simulink model "BimanualCarvingModifiedSnapshot"  (R2013a)
settings: Solver=ode4  SolverMode=SingleTasking  StartTime=0.0  StopTime=inf  FixedStep=0.0005  RelTol=1e-3
StartFcn:
  |  warndlg('Dexterit-E models cannot run under simulation. Please compile your model and run it from within Dexterit-E.');set_param(bdroot,'SimulationCommand','stop')
model workspace (MAT data in the model file):
  BKIN_STEP_TIME = 0.0005
  col_x = 1
  col_y = 2
  WIDTH = 3
  HEIGHT = 4
  TARGET_COL = 1
  LOAD = 2
  TRAJ_DURATION_COL = 3
  MAX_LOAD = 2
  FORCE_ON = 1
  HAND_RADIUS = 6
  REST_COL = 4
  TRAINING_COL = 5
  HAND_COLOR = 5
  TARGET_STROKE = 8
  TARGET_RADIUS = 9
  xMaxCursor = 15
  yMaxCursor = 16
  TARGET_COLOR = 7
  START_X = 10
  START_Y = 11
  STIFFNESS_MATERIAL = 3
  MATERIAL_MASS = 4
  MATERIAL_DAMPING = 5
  STIFFNESS_HANDS = 6
  MATERIAL_GOAL_COLOR = 12
  SCALE_VIBRATION = 7
  STONE_WIDTH = 6
  MATERIAL_DUCTILITY = 8
  TARG_COLOR = 1
  TEXT_COLOR = 13
  TEXTBOX_WIDTH = 14
  TEXTBOX_HEIGHT = 15
  ROTATION = 16
  LABEL_TEXT = 17
  LABEL_COLOR = 18
  LABEL_HEIGHT = 19
  ADVANCE_EMG_PLACEMENT = 2
  ADVANCE_EMG_MAX = 3
  EMG_ADVANCE_BUTTON = 1
  EMG_MVC_BUTTON = 2
  START_TRIAL = 3
  END_TRIAL = 4
  MUSC_NUM = 2
  HAND_DISTANCE = 3
  SYN_NUM = 4
undefined symbols (not defined in the file or in its folder): slselsubs
libraries: xpclib x9, simulink x6, General x3, KINARM_loads x2, Video x2, KINARM_IO x1, KINARM_EP_loads x1
(part 3 of 6)

== matlab function BimanualCarvingModifiedSnapshot/Draw_Hand_Endpoint/MATLAB Function ==
  data: target input; VCODE output; state_in input; target_type input; opacity_in input; target_display input; x_index input; y_index input; num_states input; stateindices input; target_labels input; KINData input; trial_state input
function VCODE = fcn(target, state_in, target_type, opacity_in, target_display, x_index, y_index, num_states, stateindices, target_labels, KINData, trial_state)

% stateindices should follow this order (depending on target-type):
% 1: length of tool (m)
% 2: stroke colour
% 3: stroke width
% 4: major radius / radius / start point (line)
% 5: minor radius / end point (line)
% 6: orientation angle



% VCODEs are length 70. All units in a VCODE should be SI, e.g. (m) and (rad). Elements in a VCODE are defined as follows:
%
% For all target types:
%  1: target type
%       1 - circle
%       2 - ellipse
%       3 - rectangle
%       4 - line
%       5 - triangle
%       11 - circle with label
%       12 - ellipse with label
%       13 - rectangle with label
%       14 - line with label
%       15 - triangle with label
%  2: target on/off status and target display (which display target will appear on)
%		0 - off
%		1 - on, appearing on both subject and operator displays
%       2 - on, appearing on subject display only
%       3 - on, appearing on operator display only
%  3: x position (m)
%  4: y position (m)
%  5: fill colour (RRGGBB) or texture index
%  6: stroke colour (RRGGBB) or texture index
%  7: stroke width
%  8: reserved for target background ID
%  9: opacity
%
% For circles:
%  10: radius (m)
%
% For ellipses:
%  10: major radius (m)
%  11: minor radius (m)
%  12: orientation of major axis (rad)
%
% For rectangles:
%  10: length (m)
%  11: height (m)
%  12: orientation (rad) (relative to x, y already shown)
%
% For lines:
%  10: endpoint x-axis coordinate relative to start point (m)
%  11: endpoint y-axis coordinate relative to start point (m)
%
% For triangles:
%  10: length (m)
%  11: height (m)
%  12: offset of peak from midpoint of length (m)
%  13: orientation (rad)
%
% For all labelled target types:
%  14: reserved
%  15-64: label characters (indexes in ISO 8859-1 character set)
%  65: label colour (0xRRGGBB), opacity is set by the vcode's opacity (9).
%  66: label height (m)
%  67: reserved
%  68: reserved
%  69: reserved
%  70: reserved

num_targets = 2;

% NOTE: we assume that the STATE and/or OPACITY inputs are vectors. 

% If the length of the input STATE is not the same as the number of targets then make STATE a column vector of the same length as 
% the TARGET input, using the first STATE (i.e. all targets get the same state) 
if num_targets == length(state_in)
	state = reshape(state_in, num_targets, 1);
else
	state = state_in(1) * ones(num_targets, 1);
end


% If the length of the input OPACITY is not the same as the number of targets then make OPACITY a column vector of the same length as
% the TARGET input, using the first OPACITY (i.e. all targets get the same opacity) 
if num_targets == length(opacity_in)
	opacity = reshape(opacity_in, num_targets, 1);
else
	opacity = opacity_in(1) * ones(num_targets, 1);
end


% Clamping the opacity to [0, 100].
opacity = min(opacity, 100);
opacity = max(opacity, 0);

VCODE = zeros(num_targets, 70);

% Set the target type. Targets with labels have type codes 10 greater than their unlabelled counterparts.
VCODE(:, 1) = target_type + 10;

% Set the hand position for both arms
VCODE(1, 3) = KINData(1,23);  % x position (m)
VCODE(1, 4) = KINData(1,24);  % y position (m)
VCODE(2, 3) = KINData(2,23);  % x position (m)
VCODE(2, 4) = KINData(2,24);  % y position (m)


for ii = 1:num_targets
	% Set the target on/off state. If the state input is 0, the target is off. Users of the VCODE should respect this
	% as an indication that the rest of the VCODE will be uninitialized.
	if (state(1) <= 0) || (state(1) > num_states)
		VCODE(ii, 2) = 0;  % target is off
	else
		VCODE(ii, 2) = target_display;  % Default is that target is on; target displays as specified by block mask
	end

	fill_colour_col = stateindices(state(1), 1);
	stroke_colour_col = stateindices(state(1), 2);
	stroke_width_col = stateindices(state(1), 3);
	
	% Set the fill colour. Fill colour currently comes from the GUI in RRRGGGBBB format.
	if fill_colour_col == 0
		VCODE(ii, 5) = -2^31;
	elseif target(fill_colour_col) < 0
		VCODE(ii, 5) = target(1, fill_colour_col);
	else
		VCODE(ii, 5) = colourshift(target(1, fill_colour_col));
    end
    if trial_state==1
        VCODE(ii,5) = colourshift(1000000000);
    end

	
	% Set the stroke colour. Stroke colour currently comes from the GUI in RRRGGGBBB format.
	if stroke_colour_col == 0
		VCODE(ii, 6) = -2^31;
	elseif target(stroke_colour_col) < 0
		VCODE(ii, 6) = target(1, stroke_colour_col);
	else
		VCODE(ii, 6) = colourshift( target(1, stroke_colour_col) );
    end
    VCODE(ii,6) = colourshift(1000000000);

	% Set the stroke width. if target table index for stroke width is zero, then the stroke width is undefined
	if stroke_width_col == 0
		VCODE(ii, 7) = 0;                   % if stroke width column is 0, then stroke width is 0
	elseif stroke_width_col < 0
		VCODE(ii, 7) = 0.001;               % if stroke width column is -ve, then a 1mm default is chosen
	else
		VCODE(ii, 7) = target(1, stroke_width_col) * 0.01;  % if stroke width column is +ve, convert width from (cm) in target table to (m)
	end

	% Set the opacity value
	VCODE(ii, 9) = 100;

	% Set attributes specific to each target type. In the process, note the first state vector column used for label information.
	label_index = 1;

	% Set attributes specific to each target type.
	if target_type == 1

		% Handle circle target:
		radius_col = stateindices(state(1), 4);
		VCODE(ii, 10)=target(1, radius_col);  % radius (convert from (cm) in target table to (m))
	    label_index = 5;

	elseif target_type == 2 || target_type == 3

	    % Handle ellipse or rectangle target:
		major_col = stateindices(state(ii), 4);
		minor_col = stateindices(state(ii), 5);
		orientation_col = stateindices(state(ii), 6);
		
		VCODE(ii, 10) = target(ii, major_col) * 0.01;  % major radius (convert from (cm) in target table to (m))
		VCODE(ii, 11) = target(ii, minor_col) * 0.01;  % minor radius (convert from (cm) in target table to (m))
		if orientation_col == 0
			VCODE(ii, 12) = 0;  % if orientation column is 0, set orientation to 0 rad
		else
			VCODE(ii, 12) = mod(target(ii, orientation_col), 360) * pi / 180.0;  % orientation (convert from (degrees) in target table to (rad))
		end
	    label_index = 7;
	
	elseif target_type == 4

		% Handle line target:
		%xendpoint_col = stateindices(state(ii), 4);
		%yendpoint_col = stateindices(state(ii), 5);
		VCODE(ii, 10) = 0;  % line endpoint in x axis, relative to start (m)
		VCODE(ii, 11) = stateindices(state(ii), 1);  % line endpoint in y axis, relative to start (taken from Target Table)
	    label_index = 6;

	elseif target_type == 5

		% Handle triangle target:
		length_col = stateindices(state(ii), 4);
		height_col = stateindices(state(ii), 5);
		offset_col = stateindices(state(ii), 6);
		orientation_col = stateindices(state(ii), 7);

		VCODE(ii, 10) = target(ii, length_col) * 0.01;  % length (convert from (cm) in target table to (m))

		% If the height column is set to 0 then the triangle is automatically made equilateral, with the base length used as length
		% for all sides. If the height column is non-zero, separate values for height and peak offset are taken from the target table.
		if height_col == 0
			VCODE(ii, 11) = sin(pi / 3.0) * VCODE(ii, 10);  % height for equilateral triangle
			VCODE(ii, 12) = 0;                          % peak offset for equilateral triangle
		else
			VCODE(ii, 11) = target(ii, height_col) * 0.01;  % height (convert from (cm) in target table to (m))
			VCODE(ii, 12) = target(ii, offset_col) * 0.01;  % peak offset (convert from (cm) in target table to (m))
		end

		if orientation_col == 0
			VCODE(ii, 13) = 0;  % if orientation column is 0, set orientation to 0 rad
		else
			VCODE(ii, 13) = mod(target(ii, orientation_col), 360) * pi / 180.0;  % orientation (convert from (degrees) in target table to (rad))
		end
	    label_index = 8;
		
	end
	%{
	% Copy the label characters to the VCODE.
	for jj = 1:50
		VCODE(ii, jj + 14) = target_labels( target( ii, stateindices(state(ii), label_index) ), jj );
	end

	% Set the label colour. Like other colours, label colour comes from the GUI in RRRGGGBBB format and is converted to a 32-bit
	% 0xRRGGBB value here. If the target column table index for the colour is 0, the label is transparent.
	if stateindices(state(ii), label_index + 1) == 0
		VCODE(ii, 65) = -2^31;
	elseif target( ii, stateindices(state(ii), label_index + 1) ) < 0
		VCODE(ii, 65) = target( ii, stateindices(state(ii), label_index + 1) );
	else
		VCODE(ii, 65) = colourshift( target( ii, stateindices(state(ii), label_index + 1) ) );
	end

	% Set the label height. Label height is converted from (cm) in the target table to (m).
	VCODE(ii, 66) = target( ii, stateindices(state, label_index + 2) ) * 0.01;
    %}

	
end

% The colourshift function converts an "RRRGGGBBB" colour value to RRGBB (as an uint32).
function RRGGBBAA = colourshift(RRRGGGBBB)

%this is "no fill"
if RRRGGGBBB == 1000000000
    RRGGBBAA = cast(16777216, 'uint32'); %hex 0x1000000
    return; 
end

blue = cast(mod(RRRGGGBBB, 1000), 'uint32');
green = cast(mod(RRRGGGBBB - blue, 1000000) / 1000, 'uint32');
red = cast((RRRGGGBBB - (green * 1000) - blue) / 1000000, 'uint32');

RRGGBBAA = bitshift(red, 16) + bitshift(green, 8) + blue;

== matlab function BimanualCarvingModifiedSnapshot/MATLAB Function1 ==
  data: SET_EXP_PARAMS1 input; HandAtStart output; KINdata input; hand_distance input; HandAtFinish output; xStart output; yStart output; HandVelXR output; HandVelYR output; HandVelXL output; HandVelYL output; HandDistance output; yFinish output
function [HandAtStart,HandAtFinish,xStart,yStart,HandVelXR,HandVelYR,HandVelXL,HandVelYL,HandDistance,yFinish] = Hand_at_start(SET_EXP_PARAMS1, KINdata,hand_distance)

% Position of robot during whole task
xStart = SET_EXP_PARAMS1(1);
yStart = SET_EXP_PARAMS1(2);

% Start and end radius of movement
StartRadius = SET_EXP_PARAMS1(5);

% Distance between hands
% HandDistance = 0.15;%0.22;%HAND_DISTANCE;
HandDistance = hand_distance;

% Finish line
yFinish = 0.08;

% % Check to see if hand or tool endpoint is in target
% HandPosX = KINdata(1,23);
% HandPosY = KINdata(1,24);
% HandVelX = KINdata(1,25);
% HandVelY = KINdata(1,26);

% Is hand inside (xInit,yInit)?
% HandAtStart = double(sqrt((HandPosX-xStart)^2+(HandPosY-yStart)^2)<StartRadius);

% Check to see if hand or tool endpoint is in target
HandPosXR = KINdata(1,23);
HandPosYR = KINdata(1,24);
HandVelXR = KINdata(1,25);
HandVelYR = KINdata(1,26);
HandPosXL = KINdata(2,23);
HandPosYL = KINdata(2,24);
HandVelXL = KINdata(2,25);
HandVelYL = KINdata(2,26);

% Is hand inside (xInit,yInit)?
HandAtStart = double(sqrt((HandPosXR-(xStart+HandDistance/2))^2+(HandPosYR-yStart)^2)<StartRadius  && sqrt((HandPosXL-(xStart-HandDistance/2))^2+(HandPosYL-yStart)^2)<StartRadius);
% User wants to finish?
HandAtFinish = double(HandPosYR<yFinish  && HandPosYL<yFinish);

== matlab function BimanualCarvingModifiedSnapshot/Draw_finish_line/MATLAB Function ==
  data: target input; VCODE output; state_in input; target_type input; opacity_in input; target_display input; x_index input; y_index input; num_states input; stateindices input; target_labels input; KINData input; yWall input; trial_state input
function VCODE = fcn(target, state_in, target_type, opacity_in, target_display, x_index, y_index, num_states, stateindices, target_labels, KINData, yWall, trial_state)

% stateindices should follow this order (depending on target-type):
% 1: fill colour
% 2: stroke colour
% 3: stroke width
% 4: major radius / radius / start point (line)
% 5: minor radius / end point (line)
% 6: orientation angle



% VCODEs are length 70. All units in a VCODE should be SI, e.g. (m) and (rad). Elements in a VCODE are defined as follows:
%
% For all target types:
%  1: target type
%       1 - circle
%       2 - ellipse
%       3 - rectangle
%       4 - line
%       5 - triangle
%       11 - circle with label
%       12 - ellipse with label
%       13 - rectangle with label
%       14 - line with label
%       15 - triangle with label
%  2: target on/off status and target display (which display target will appear on)
%		0 - off
%		1 - on, appearing on both subject and operator displays
%       2 - on, appearing on subject display only
%       3 - on, appearing on operator display only
%  3: x position (m)
%  4: y position (m)
%  5: fill colour (RRGGBB) or texture index
%  6: stroke colour (RRGGBB) or texture index
%  7: stroke width
%  8: reserved for target background ID
%  9: opacity
%
% For circles:
%  10: radius (m)
%
% For ellipses:
%  10: major radius (m)
%  11: minor radius (m)
%  12: orientation of major axis (rad)
%
% For rectangles:
%  10: length (m)
%  11: height (m)
%  12: orientation (rad) (relative to x, y already shown)
%
% For lines:
%  10: endpoint x-axis coordinate relative to start point (m)
%  11: endpoint y-axis coordinate relative to start point (m)
%
% For triangles:
%  10: length (m)
%  11: height (m)
%  12: offset of peak from midpoint of length (m)
%  13: orientation (rad)
%
% For all labelled target types:
%  14: reserved
%  15-64: label characters (indexes in ISO 8859-1 character set)
%  65: label colour (0xRRGGBB), opacity is set by the vcode's opacity (9).
%  66: label height (m)
%  67: reserved
%  68: reserved
%  69: reserved
%  70: reserved

num_targets = 1;

% NOTE: we assume that the STATE and/or OPACITY inputs are vectors. 

% If the length of the input STATE is not the same as the number of targets then make STATE a column vector of the same length as 
% the TARGET input, using the first STATE (i.e. all targets get the same state)
if num_targets == length(state_in)
	state = reshape(state_in, num_targets, 1);
else
	state = state_in(1) * ones(num_targets, 1);
end


% If the length of the input OPACITY is not the same as the number of targets then make OPACITY a column vector of the same length as
% the TARGET input, using the first OPACITY (i.e. all targets get the same opacity)
if num_targets == length(opacity_in)
	opacity = reshape(opacity_in, num_targets, 1);
else
	opacity = opacity_in(1) * ones(num_targets, 1);
end


% Clamping the opacity to [0, 100].
opacity = min(opacity, 100);
opacity = max(opacity, 0);

VCODE = zeros(num_targets, 70);

% Set the target type. Targets with labels have type codes 10 greater than their unlabelled counterparts.
VCODE(:, 1) = target_type + 10;
VCODE(:, 2) = target_display;

VCODE(:, 5) = colourshift(target(1, stateindices(state(1), 1)));
VCODE(:, 6) = colourshift(target(1, stateindices(state(1), 1)));

% Set the opacity value
VCODE(:, 9) = opacity_in(1);
% Target only visible during tracking in trial_state==2
if trial_state==0
    VCODE(:, 5) = colourshift(1000000000);
    VCODE(:, 6) = colourshift(1000000000);
    VCODE(:, 9) = 0;
end


% Stroke width
VCODE(:, 7) = target(1, stateindices(state(1), 3))*0.01 * 2 / 3;

VCODE(:, 3) = -0.5;  % x position (m)
VCODE(:, 4) = yWall;  % y position (m)

VCODE(:, 10) = 1;  % line endpoint in x axis, relative to start (m)
VCODE(:, 11) = 0;  % line endpoint in y axis, relative to start (m)

%{
persistent TargetIndex;
if isempty(TargetIndex), TargetIndex = 1; end
% Set the hand position.
if TargetIndex<=length(xMaterial)
    % Initially draw the whole material from left to right
    % Line beginning
    VCODE(:, 3) = xMaterial(TargetIndex);  % x position (m)
    VCODE(:, 4) = yMaterial(TargetIndex);  % y position (m)
    
    % Line endpoint
    VCODE(:, 10) = xMaterial(TargetIndex+1)-VCODE(:,3);  % line endpoint in x axis, relative to start (m)
    VCODE(:, 11) = yMaterial(TargetIndex+1)-VCODE(:,4);  % line endpoint in y axis, relative to start (m)
else
    % After material is all drawn, update only the changing section
    % Line beginning
    VCODE(:, 3) = xMaterial(MaterialUpdateInd1);  % x position (m)
    VCODE(:, 4) = yMaterial(MaterialUpdateInd1);  % y position (m)
    
    % Line endpoint
    VCODE(:, 10) = xMaterial(MaterialUpdateInd2)-VCODE(:,3);  % line endpoint in x axis, relative to start (m)
    VCODE(:, 11) = yMaterial(MaterialUpdateInd2)-VCODE(:,4);  % line endpoint in y axis, relative to start (m)
end


TargetIndex = min(length(xMaterial)+5,TargetIndex+1);
%}
%{
for ii = 1:num_targets
	% Set the target on/off state. If the state input is 0, the target is off. Users of the VCODE should respect this
	% as an indication that the rest of the VCODE will be uninitialized.
	if (state(ii) <= 0) || (state(ii) > num_states)
		VCODE(ii, 2) = 0;  % target is off
	else
		VCODE(ii, 2) = target_display;  % Default is that target is on; target displays as specified by block mask
	end

	fill_colour_col = stateindices(state(ii), 1);
	stroke_colour_col = stateindices(state(ii), 2);
	stroke_width_col = stateindices(state(ii), 3);
	
	% Set the fill colour. Fill colour currently comes from the GUI in RRRGGGBBB format.
	%{
    if fill_colour_col == 0
		VCODE(ii, 5) = -2^31;
	elseif target(fill_colour_col) < 0
		VCODE(ii, 5) = target(ii, fill_colour_col);
	else
		VCODE(ii, 5) = colourshift(target(ii, fill_colour_col));
    end
    %}
    VCODE(ii,5) = colourshift(1000000000);
	
	% Set the stroke colour. Stroke colour currently comes from the GUI in RRRGGGBBB format.
    if trial_state==1
        if stroke_colour_col == 0
            VCODE(ii, 6) = -2^31;
        elseif target(stroke_colour_col) < 0
            VCODE(ii, 6) = target(ii, stroke_colour_col);
        else
            VCODE(ii, 6) = colourshift( target(ii, stroke_colour_col) );
        end
    else
        % CIRCLE APPEARS ONLY DURING TASK
        VCODE(ii, 6) = colourshift(1000000000);
    end

	% Set the stroke width. if target table index for stroke width is zero, then the stroke width is undefined
	if stroke_width_col == 0
		VCODE(ii, 7) = 0;                   % if stroke width column is 0, then stroke width is 0
	elseif stroke_width_col < 0
		VCODE(ii, 7) = 0.001;               % if stroke width column is -ve, then a 1mm default is chosen
	else
		VCODE(ii, 7) = target(ii, stroke_width_col) * 0.01;  % if stroke width column is +ve, convert width from (cm) in target table to (m)
    end

	% Set the opacity value
	VCODE(ii, 9) = opacity(ii);

	% Set attributes specific to each target type. In the process, note the first state vector column used for label information.
	label_index = 1;

	% Set attributes specific to each target type.
	if target_type == 1

		% Handle circle target:
		radius_col = stateindices(state(ii), 4);
		VCODE(ii, 10)=target(ii, radius_col);  % radius (in m)
	    label_index = 5;

	elseif target_type == 2 || target_type == 3

	    % Handle ellipse or rectangle target:
		major_col = stateindices(state(ii), 4);
		minor_col = stateindices(state(ii), 5);
		orientation_col = stateindices(state(ii), 6);
		
		VCODE(ii, 10) = target(ii, major_col) * 0.01;  % major radius (convert from (cm) in target table to (m))
		VCODE(ii, 11) = target(ii, minor_col) * 0.01;  % minor radius (convert from (cm) in target table to (m))
		if orientation_col == 0
			VCODE(ii, 12) = 0;  % if orientation column is 0, set orientation to 0 rad
		else
			VCODE(ii, 12) = mod(target(ii, orientation_col), 360) * pi / 180.0;  % orientation (convert from (degrees) in target table to (rad))
		end
	    label_index = 7;
	
	elseif target_type == 4

		% Handle line target:
		%xendpoint_col = stateindices(state(ii), 4);
		%yendpoint_col = stateindices(state(ii), 5);
		VCODE(ii, 10) = 0;  % line endpoint in x axis, relative to start (m)
		VCODE(ii, 11) = stateindices(state(ii), 1);  % line endpoint in y axis, relative to start (taken from Target Table)
	    label_index = 6;

	elseif target_type == 5

		% Handle triangle target:
		length_col = stateindices(state(ii), 4);
		height_col = stateindices(state(ii), 5);
		offset_col = stateindices(state(ii), 6);
		orientation_col = stateindices(state(ii), 7);

		VCODE(ii, 10) = target(ii, length_col) * 0.01;  % length (convert from (cm) in target table to (m))

		% If the height column is set to 0 then the triangle is automatically made equilateral, with the base length used as length
		% for all sides. If the height column is non-zero, separate values for height and peak offset are taken from the target table.
		if height_col == 0
			VCODE(ii, 11) = sin(pi / 3.0) * VCODE(ii, 10);  % height for equilateral triangle
			VCODE(ii, 12) = 0;                          % peak offset for equilateral triangle
		else
			VCODE(ii, 11) = target(ii, height_col) * 0.01;  % height (convert from (cm) in target table to (m))
			VCODE(ii, 12) = target(ii, offset_col) * 0.01;  % peak offset (convert from (cm) in target table to (m))
		end

		if orientation_col == 0
			VCODE(ii, 13) = 0;  % if orientation column is 0, set orientation to 0 rad
		else
			VCODE(ii, 13) = mod(target(ii, orientation_col), 360) * pi / 180.0;  % orientation (convert from (degrees) in target table to (rad))
		end
	    label_index = 8;
		
	end
	
	% Copy the label characters to the VCODE.
	for jj = 1:50
		VCODE(ii, jj + 14) = target_labels( target( ii, stateindices(state(ii), label_index) ), jj );
	end

	% Set the label colour. Like other colours, label colour comes from the GUI in RRRGGGBBB format and is converted to a 32-bit
	% 0xRRGGBB value here. If the target column table index for the colour is 0, the label is transparent.
	if stateindices(state(ii), label_index + 1) == 0
		VCODE(ii, 65) = -2^31;
	elseif target( ii, stateindices(state(ii), label_index + 1) ) < 0
		VCODE(ii, 65) = target( ii, stateindices(state(ii), label_index + 1) );
	else
		VCODE(ii, 65) = colourshift( target( ii, stateindices(state(ii), label_index + 1) ) );
	end

	% Set the label height. Label height is converted from (cm) in the target table to (m).
	VCODE(ii, 66) = target( ii, stateindices(state, label_index + 2) ) * 0.01;


	
end
%}
% The colourshift function converts an "RRRGGGBBB" colour value to RRGBB (as an uint32).
function RRGGBBAA = colourshift(RRRGGGBBB)

%this is "no fill"
if RRRGGGBBB == 1000000000
    RRGGBBAA = cast(16777216, 'uint32'); %hex 0x1000000
    return; 
end

blue = cast(mod(RRRGGGBBB, 1000), 'uint32');
green = cast(mod(RRRGGGBBB - blue, 1000000) / 1000, 'uint32');
red = cast((RRRGGGBBB - (green * 1000) - blue) / 1000000, 'uint32');

RRGGBBAA = bitshift(red, 16) + bitshift(green, 8) + blue;

== matlab function BimanualCarvingModifiedSnapshot/emgScoreVCode ==
  settings: fimath=|
      | fimath(...
      | 'RoundMode', 'floor',...
      | 'OverflowMode', 'wrap',...
      | 'ProductMode', 'KeepLSB', 'ProductWordLength', 32,...
      | 'SumMode', 'KeepLSB', 'SumWordLength', 32,...
      | 'CastBeforeSum', false)
  data: VCODE input; VCODE_out output; emgBuffer input; residualBuffer input; R2 output; smoothnessScore input
function [VCODE_out,R2] = emgScoreVCode(VCODE, emgBuffer, residualBuffer,smoothnessScore)

persistent R2Buffer;
if isempty(R2Buffer); R2Buffer = zeros(1,200); end

sse = sum(residualBuffer);
sst = sum(sum((emgBuffer - mean(mean(emgBuffer))).^2));
R2_value = 100*(1 - sse/sst);

R2Buffer = [R2_value R2Buffer(:,1:end-1)];

R2 = mean(R2Buffer);
% R2 = smoothnessScore*1e7;

%don't show a zero, show a blank in the 100's position
if R2 < 100
	VCODE(15) = 32; %' ' space
else
	VCODE(15) = getChar(R2, 100);
end

%don't show a zero, show a blank in the 10's position
if R2 < 10
	VCODE(16) = 32; %' ' space
else
	VCODE(16) = getChar(R2, 10);
end

VCODE(17) = getChar(R2, 1);
VCODE(18) = 0;
% VCODE(18) = 46; % . period
% VCODE(19) = getChar(R2, 0.1);
% VCODE(20) = 0;	 %terminate the new string
% VCODE(20) = 32;  %' ' space
% VCODE(19) = 99;  % c
% VCODE(20) = 109; % m
% VCODE(21) = 47;  % \
% VCODE(22) = 115; % s

VCODE_out=VCODE;
end

function cc = getChar(number, dec)
	%in simulink there is no nice way to convert a number to s string
	%so what we are doing here is converting a single digit to a character.
	%48 is ascii for '0', so this gets the least significant digit before 
	%the decimal and converts to ascii.
    cc = floor(mod(number / dec, 10)) + 48;
end

== matlab function BimanualCarvingModifiedSnapshot/sample_buffer ==
  data: resid_sample input; res_history output; d_sample input; d_history output
function [res_history,d_history] = sample_buffer(resid_sample,d_sample)
%#codegen

persistent res d;
if isempty(res); res = zeros(1,100); end
if isempty(d); d = zeros(16,100); end

ss_resid = sum(resid_sample.^2);
res = [ss_resid res(:,1:end-1)];
d = [d_sample d(:,1:end-1)];

res_history = res;
d_history = d;

end

== matlab function BimanualCarvingModifiedSnapshot/EMG Processing/MATLAB Function1 ==
  data: emg input; memg output; measure_min_emg input
function memg = measure_minimum_emg(emg,measure_min_emg)

persistent min_emg nsamp measuring;
if isempty(min_emg); min_emg = zeros(size(emg)); end
if isempty(nsamp); nsamp = 0; end
if isempty(measuring); measuring = 0; end

if ~measure_min_emg
    measuring = 0;
else
    if ~measuring
        min_emg = zeros(size(emg));
        nsamp = 0;
        measuring = 1;    
    else
        nsamp = nsamp + 1;
        min_emg = min_emg + (1/(nsamp + 1))*(emg - min_emg);
    end
end

memg = zeros(size(emg));
% memg = min_emg;
end

== matlab function BimanualCarvingModifiedSnapshot/Draw_message/MATLAB Function ==
  data: target input; VCODE output; state_in input; target_type input; opacity_in input; target_display input; x_index input; y_index input; num_states input; stateindices input; target_labels input; KINData input; xInit input; yInit input; trial_state input
function VCODE = fcn(target, state_in, target_type, opacity_in, target_display, x_index, y_index, num_states, stateindices, target_labels, KINData, xInit,yInit,trial_state)

% stateindices should follow this order (depending on target-type):
% 1: length of tool (m)
% 2: stroke colour
% 3: stroke width
% 4: major radius / radius / start point (line)
% 5: minor radius / end point (line)
% 6: orientation angle



% VCODEs are length 70. All units in a VCODE should be SI, e.g. (m) and (rad). Elements in a VCODE are defined as follows:
%
% For all target types:
%  1: target type
%       1 - circle
%       2 - ellipse
%       3 - rectangle
%       4 - line
%       5 - triangle
%       11 - circle with label
%       12 - ellipse with label
%       13 - rectangle with label
%       14 - line with label
%       15 - triangle with label
%  2: target on/off status and target display (which display target will appear on)
%		0 - off
%		1 - on, appearing on both subject and operator displays
%       2 - on, appearing on subject display only
%       3 - on, appearing on operator display only
%  3: x position (m)
%  4: y position (m)
%  5: fill colour (RRGGBB) or texture index
%  6: stroke colour (RRGGBB) or texture index
%  7: stroke width
%  8: reserved for target background ID
%  9: opacity
%
% For circles:
%  10: radius (m)
%
% For ellipses:
%  10: major radius (m)
%  11: minor radius (m)
%  12: orientation of major axis (rad)
%
% For rectangles:
%  10: length (m)
%  11: height (m)
%  12: orientation (rad) (relative to x, y already shown)
%
% For lines:
%  10: endpoint x-axis coordinate relative to start point (m)
%  11: endpoint y-axis coordinate relative to start point (m)
%
% For triangles:
%  10: length (m)
%  11: height (m)
%  12: offset of peak from midpoint of length (m)
%  13: orientation (rad)
%
% For all labelled target types:
%  14: reserved
%  15-64: label characters (indexes in ISO 8859-1 character set)
%  65: label colour (0xRRGGBB), opacity is set by the vcode's opacity (9).
%  66: label height (m)
%  67: reserved
%  68: reserved
%  69: reserved
%  70: reserved

num_targets = size(target, 1);

% NOTE: we assume that the STATE and/or OPACITY inputs are vectors. 

% If the length of the input STATE is not the same as the number of targets then make STATE a column vector of the same length as 
% the TARGET input, using the first STATE (i.e. all targets get the same state) 
if num_targets == length(state_in)
	state = reshape(state_in, num_targets, 1);
else
	state = state_in(1) * ones(num_targets, 1);
end


% If the length of the input OPACITY is not the same as the number of targets then make OPACITY a column vector of the same length as
% the TARGET input, using the first OPACITY (i.e. all targets get the same opacity)
if num_targets == length(opacity_in)
	opacity = reshape(opacity_in, num_targets, 1);
else
	opacity = opacity_in(1) * ones(num_targets, 1);
end


% Clamping the opacity to [0, 100].
opacity = min(opacity, 100);
opacity = max(opacity, 0);

VCODE = zeros(num_targets, 70);

% Set the target type. Targets with labels have type codes 10 greater than their unlabelled counterparts.
VCODE(:, 1) = target_type + 10;

% Set the hand position.
VCODE(:, 3) = xInit;  % x position (m)
VCODE(:, 4) = yInit+0.1;  % y position (m)

for ii = 1:num_targets
	% Set the target on/off state. If the state input is 0, the target is off. Users of the VCODE should respect this
	% as an indication that the rest of the VCODE will be uninitialized.
	if (state(ii) <= 0) || (state(ii) > num_states)
		VCODE(ii, 2) = 0;  % target is off
	else
		VCODE(ii, 2) = target_display;  % Default is that target is on; target displays as specified by block mask
	end

	fill_colour_col = stateindices(state(ii), 1);
	stroke_colour_col = stateindices(state(ii), 2);
	stroke_width_col = stateindices(state(ii), 3);
	
	% Set the fill colour. Fill colour currently comes from the GUI in RRRGGGBBB format.
	if fill_colour_col == 0
		VCODE(ii, 5) = -2^31;
	elseif target(fill_colour_col) < 0
		VCODE(ii, 5) = target(ii, fill_colour_col);
	else
		VCODE(ii, 5) = colourshift(target(ii, fill_colour_col));
	end
	
	% Set the stroke colour. Stroke colour currently comes from the GUI in RRRGGGBBB format.
	if stroke_colour_col == 0
		VCODE(ii, 6) = -2^31;
	elseif target(stroke_colour_col) < 0
		VCODE(ii, 6) = target(ii, stroke_colour_col);
	else
		VCODE(ii, 6) = colourshift( target(ii, stroke_colour_col) );
	end

	% Set the stroke width. if target table index for stroke width is zero, then the stroke width is undefined
	if stroke_width_col == 0
		VCODE(ii, 7) = 0;                   % if stroke width column is 0, then stroke width is 0
	elseif stroke_width_col < 0
		VCODE(ii, 7) = 0.001;               % if stroke width column is -ve, then a 1mm default is chosen
	else
		VCODE(ii, 7) = target(ii, stroke_width_col) * 0.01;  % if stroke width column is +ve, convert width from (cm) in target table to (m)
    end

    VCODE(ii,5) = colourshift(1000000000);
    VCODE(ii,6) = colourshift(1000000000);
    VCODE(ii,7) = colourshift(1000000000);
    
	% Set the opacity value
    %if trial_state==1 || trial_state==2
    %    VCODE(ii, 9) = 0;
    %else
        VCODE(ii, 9) = opacity(ii);
    %end

	% Set attributes specific to each target type. In the process, note the first state vector column used for label information.
	label_index = 1;

	% Set attributes specific to each target type.
	if target_type == 1

		% Handle circle target:
		radius_col = stateindices(state(ii), 4);
		VCODE(ii, 10)=target(ii, radius_col) * 0.01;  % radius (convert from (cm) in target table to (m))
	    label_index = 5;

	elseif target_type == 2 || target_type == 3

	    % Handle ellipse or rectangle target:
		major_col = stateindices(state(ii), 4);
		minor_col = stateindices(state(ii), 5);
		orientation_col = 0;%stateindices(state(ii), 6);
		
		VCODE(ii, 10) = target(ii, major_col)*15;  % major radius (convert from (cm) in target table to (m))
		VCODE(ii, 11) = target(ii, minor_col)*15;  % minor radius (convert from (cm) in target table to (m))
		if orientation_col == 0
			VCODE(ii, 12) = 0;  % if orientation column is 0, set orientation to 0 rad
		else
			VCODE(ii, 12) = mod(target(ii, orientation_col), 360) * pi / 180.0;  % orientation (convert from (degrees) in target table to (rad))
		end
	    label_index = 7;
	
	elseif target_type == 4

		% Handle line target:
		xendpoint_col = stateindices(state(ii), 8);
		yendpoint_col = stateindices(state(ii), 9);
		VCODE(ii, 10) = target(ii, xendpoint_col) * 0.01;  % line endpoint in x axis, relative to start (convert from (cm) in target table to (m))
		VCODE(ii, 11) = target(ii, yendpoint_col) * 0.01;  % line endpoint in y axis, relative to start (convert from (cm) in target table to (m))
	    label_index = 6;

	elseif target_type == 5

		% Handle triangle target:
		length_col = stateindices(state(ii), 4);
		height_col = stateindices(state(ii), 5);
		offset_col = stateindices(state(ii), 6);
		orientation_col = stateindices(state(ii), 7);

		VCODE(ii, 10) = target(ii, length_col) * 0.01;  % length (convert from (cm) in target table to (m))

		% If the height column is set to 0 then the triangle is automatically made equilateral, with the base length used as length
		% for all sides. If the height column is non-zero, separate values for height and peak offset are taken from the target table.
		if height_col == 0
			VCODE(ii, 11) = sin(pi / 3.0) * VCODE(ii, 10);  % height for equilateral triangle
			VCODE(ii, 12) = 0;                          % peak offset for equilateral triangle
		else
			VCODE(ii, 11) = target(ii, height_col) * 0.01;  % height (convert from (cm) in target table to (m))
			VCODE(ii, 12) = target(ii, offset_col) * 0.01;  % peak offset (convert from (cm) in target table to (m))
		end

		if orientation_col == 0
			VCODE(ii, 13) = 0;  % if orientation column is 0, set orientation to 0 rad
		else
			VCODE(ii, 13) = mod(target(ii, orientation_col), 360) * pi / 180.0;  % orientation (convert from (degrees) in target table to (rad))
		end
	    label_index = 8;
		
	end
	
	% Copy the label characters to the VCODE.
	for jj = 1:50
		VCODE(ii, jj + 14) = target_labels( target( ii, stateindices(state(ii), label_index) ), jj );
    end

	% Set the label colour. Like other colours, label colour comes from the GUI in RRRGGGBBB format and is converted to a 32-bit
	% 0xRRGGBB value here. If the target column table index for the colour is 0, the label is transparent.
	%{
    if stateindices(state(ii), label_index + 1) == 0
		VCODE(ii, 65) = -2^31;
	elseif target( ii, stateindices(state(ii), label_index + 1) ) < 0
		VCODE(ii, 65) = target( ii, stateindices(state(ii), label_index + 1) );
	else
		VCODE(ii, 65) = colourshift( target( ii, stateindices(state(ii), 2) ) );
    end
    %}
    VCODE(ii, 65) = colourshift( target( ii, stateindices(state(ii), 2) ) );
	% Set the label height. Label height is converted from (cm) in the target table to (m).
	VCODE(ii, 66) = target( ii, stateindices(state, 5) ) * 3;


	
end



if trial_state==0 || trial_state==2
    

    
    VCODE(15) = 82; % R
    VCODE(16) = 69; % E
    VCODE(17) = 76; % L
    VCODE(18) = 65; % A
    VCODE(19) = 88; % X
    

end

end


function cc = getChar(number, dec)
	%in simulink there is no nice way to convert a number to s string
	%so what we are doing here is converting a single digit to a character.
	%48 is ascii for '0', so this gets the least significant digit before 
	%the decimal and converts to ascii.
    cc = floor(mod(number / dec, 10)) + 48;
end



% The colourshift function converts an "RRRGGGBBB" colour value to RRGBB (as an uint32).
function RRGGBBAA = colourshift(RRRGGGBBB)

%this is "no fill"
if RRRGGGBBB == 1000000000
    RRGGBBAA = cast(16777216, 'uint32'); %hex 0x1000000
    return; 
end

blue = cast(mod(RRRGGGBBB, 1000), 'uint32');
green = cast(mod(RRRGGGBBB - blue, 1000000) / 1000, 'uint32');
red = cast((RRRGGGBBB - (green * 1000) - blue) / 1000000, 'uint32');

RRGGBBAA = bitshift(red, 16) + bitshift(green, 8) + blue;

end

== matlab function BimanualCarvingModifiedSnapshot/EMG Processing/MATLAB Function2 ==
  data: emg input; maxemg output; measure_max_emg input
function maxemg = measure_maximum_emg(emg,measure_max_emg)

persistent max_emg;
if isempty(max_emg); max_emg = zeros(size(emg)); end

if measure_max_emg
    index = emg > max_emg;
    max_emg(index) = emg(index);
end

maxemg = max_emg;
end

== matlab function BimanualCarvingModifiedSnapshot/EMG Processing/MATLAB Function3 ==
  data: emg input; output_emg output; max_emg input; min_emg input; normalize input
function output_emg = output_processed_EMG(emg,max_emg,min_emg,normalize)

if normalize
    output_emg = (emg - min_emg)./(max_emg - min_emg);
else
    output_emg = emg;
end

end

== system BimanualCarvingModifiedSnapshot/Trajectory subsystem/KINARM_EP_Position_Controller/50 Hz Filter ==
  In1 : Inport
  2nd order 50Hz Butterworth{,1..3} (4 alike) : DiscreteTransferFcn  Numerator=[.0055427 .0110854 .0055427]  Denominator=[1 -1.7786318 0.8008026]  SampleTime=.0005
  Demux : Demux
  Mux : Mux
  Out1 : Outport
  wires:
  Demux/2 -> 2nd order 50Hz Butterworth1/1
  In1/1 -> Demux/1
  Mux/1 -> Out1/1
  2nd order 50Hz Butterworth1/1 -> Mux/2
  Demux/1 -> 2nd order 50Hz Butterworth/1
  2nd order 50Hz Butterworth/1 -> Mux/1
  Demux/3 -> 2nd order 50Hz Butterworth2/1
  2nd order 50Hz Butterworth2/1 -> Mux/3
  Demux/4 -> 2nd order 50Hz Butterworth3/1
  2nd order 50Hz Butterworth3/1 -> Mux/4

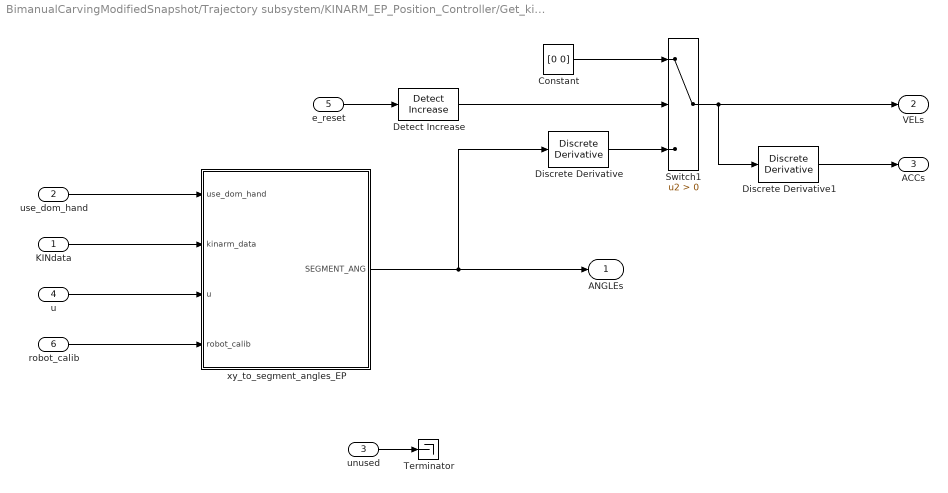
== system BimanualCarvingModifiedSnapshot/Trajectory subsystem/KINARM_EP_Position_Controller/Get_kinematics_EP ==
  KINdata : Inport
  use_dom_hand : Inport  Port=2
  unused : Inport  Port=3
  u : Inport  Port=4
  e_reset : Inport  Port=5
  robot_calib : Inport  Port=6
  Constant : Constant  Value=[0 0]
  Detect Increase : simulink/Logic and Bit Operations/Detect Increase  vinit=0.0  InputProcessing=Inherited  OutDataTypeStr=uint8
  Discrete Derivative : simulink/Discrete/Discrete Derivative  gainval=1.0  ICPrevScaledInput=0.0  InputProcessing=Inherited  OutMin=[]  OutMax=[]  OutDataType=sfix(16)  OutScaling=2^-10  DoSatur=off
  Discrete Derivative1 : simulink/Discrete/Discrete Derivative  gainval=1.0  ICPrevScaledInput=0.0  InputProcessing=Inherited  OutMin=[]  OutMax=[]  OutDataType=sfix(16)  OutScaling=2^-10  DoSatur=off
  Switch1 : Switch  Criteria=u2 > Threshold
  Terminator : Terminator
  xy_to_segment_angles_EP : MATLAB Function  TreatAsAtomicUnit=on
  ANGLEs : Outport
  VELs : Outport  Port=2
  ACCs : Outport  Port=3
  wires:
  xy_to_segment_angles_EP/1(SEGMENT_ANG) -> ANGLEs/1, Discrete Derivative/1
  Discrete Derivative/1 -> Switch1/3
  use_dom_hand/1 -> xy_to_segment_angles_EP/1(use_dom_hand)
  u/1 -> xy_to_segment_angles_EP/3(u)
  Switch1/1 -> Discrete Derivative1/1, VELs/1
  Constant/1 -> Switch1/1
  Detect Increase/1 -> Switch1/2
  Discrete Derivative1/1 -> ACCs/1
  KINdata/1 -> xy_to_segment_angles_EP/2(kinarm_data)
  e_reset/1 -> Detect Increase/1
  unused/1 -> Terminator/1
  robot_calib/1 -> xy_to_segment_angles_EP/4(robot_calib)

== stateflow chart BimanualCarvingModifiedSnapshot/Trial_Control ==
  settings: sampleTime=0.001
  state init/
    ForceOn = 0;
    minEMG_on = 0;
    maxEMG_on = 0;
    normalizeEMG_on =0;
  state EMGPlacement/
  state MVC/
    maxEMG_on = 1;
    event_code = EMG_ADVANCE_BUTTON;
  state MVC_done/
    maxEMG_on = 0;
    logging_enable = 1;
    event_code = EMG_MVC_BUTTON;
  state Main_Trial/
    state InCentre/
      normalizeEMG_on =0;
      logging_enable = 0;
      rest = Trial_Protocol[REST_COL];
      % State - wait for subject
      trial_state = 0;
      % Initialize cursor
      EMG_trigger = 0;
      ForceOn = 0;
    state StayInCentre/
      % Enable measurement of minimum EMG
      minEMG_on = 1;
    state DuringTrial/
      % Recording enabled
      logging_enable = 1;
      % Disable measurement of minimum EMG
      minEMG_on = 0;
      % Normalize EMG
      normalizeEMG_on = 1;
      % Turn force on forever
      ForceOn = 1;
      % State - during trial
      trial_state = 1;
      % Trigger
      EMG_trigger = 5;
      event_code = START_TRIAL;
    state EndOfTrial/
      logging_enable = 0;
      normalizeEMG_on = 0;
      % State - rest
      trial_state = 2;
      EMG_trigger = 0;
    StayInCentre -> InCentre [order 2] : [HandAtStart==0]
    InCentre -> StayInCentre : [HandAtStart==1]
    StayInCentre -> DuringTrial [order 1] : after(5000,e_clk)
    DuringTrial -> EndOfTrial [order 2] : [HandAtFinish==1]
    DuringTrial -> EndOfTrial [order 1] : after(Trial_Protocol[TRAJ_DURATION_COL]*1000,e_clk)
  state Inter_Trial_State/
    e_Trial_End
    event_code = END_TRIAL;
  state WaitForFlagToSet
  (default) -> init
  init -> EMGPlacement
  EMGPlacement -> MVC : e_AdvanceEMG
  MVC -> MVC_done : e_AdvanceMVC
  MVC_done -> InCentre
  Inter_Trial_State -> InCentre
  WaitForFlagToSet -> Inter_Trial_State : after(2, e_clk)
  Main_Trial -> WaitForFlagToSet : e_ExitTrialNow/
      | logging_enable = 0;
      | tickCount = 10;
  EndOfTrial -> Inter_Trial_State : after(rest*1000,e_clk)
  data: logging_enable output boolean; trial_state output double; tickCount local double; Trial_Protocol input double; HandAtStart input; rest local double; ForceOn output double; EMG_trigger output double; HandAtFinish input; minEMG_on output double; maxEMG_on output double; normalizeEMG_on output double; event_code output double
  events: e_clk input RISING_EDGE_EVENT; e_ExitTrialNow input EITHER_EDGE_EVENT; e_Trial_End output EITHER_EDGE_EVENT; e_AdvanceEMG input RISING_EDGE_EVENT; e_AdvanceMVC input RISING_EDGE_EVENT
